simulink model "RCAM_SIMULATION"  (R2024b)
settings: Solver=VariableStepAuto  StartTime=0.0  StopTime=1000  RelTol=1e-3
undefined symbols (not defined in the file or in its folder): RCAM_model
libraries: aerolibfltsims x2, aerolibatmos2 x1, aerolibanimutils x1, aerolibanim x1
Description:
  | RCAM [Research Civil Transport Aircraft Model]
  | 
  | To study the dynamic behaviour of the aircarft with te given control inputs.
  | , through the plots ang the animation plots using the real time simualtion.
settings Model: Creator=Rahul N  LastModifiedBy=rukky
settings DataIOCC: SaveTime=off  ReturnWorkspaceOutputs=off
settings ModelReferenceCC: EnableRefExpFcnMdlSchedulingChecks=on
settings RTWCC: GPUComputeCapability=3.5

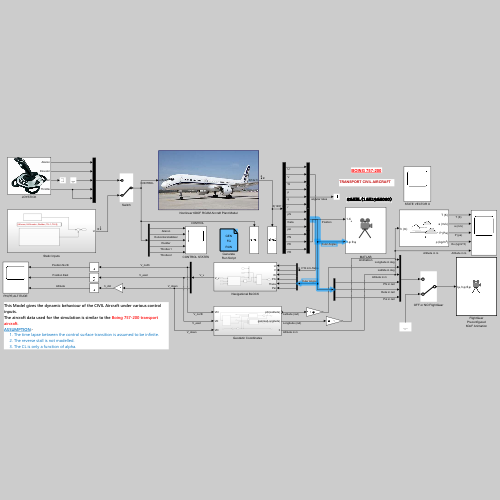
[thumbnail: Simulink's stored preview of the top-level diagram]
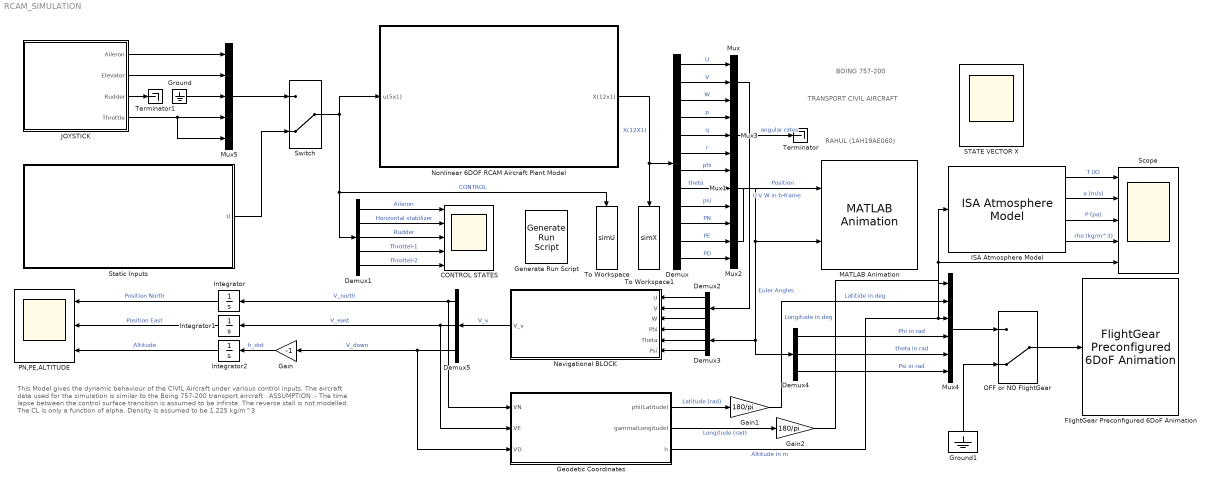
== system RCAM_SIMULATION ==
  note: RAHUL (1AH19AE060)
  note: This Model gives the dynamic behaviour of the CIVIL Aircraft under various control inputs.
      | The aircraft data used for the simulation is similar to the Boing 757-200 transport aircraft .
      | ASSUMPTION :-
      | The time lapse between the control surface transition is assumed to be infinite.
      | The reverse stall is not modelled.
      | The CL is only a function of alpha.
      | Density is assumed to be 1.225 kg/m^3
  note: TRANSPORT CIVIL AIRCRAFT
  note: BOING 757-200
  "CONTROL STATES " : Scope  NumInputPorts=5
  Demux : Demux  Outputs=12
  Demux1 : Demux  Outputs=5
  Demux{2..5} (4 alike) : Demux  Outputs=3
  FlightGear Preconfigured 6DoF Animation : aerolibfltsims/FlightGear Preconfigured 6DoF Animation  xFlightGearVersion=v2019.1  DestinationIpAddress=127.0.0.1  DestinationPort=5502  SampleTime=1/30  packetVersion=24
  Gain : Gain  Gain=-1
  Gain1 : Gain  Gain=180/pi
  Gain2 : Gain  Gain=180/pi
  Generate Run Script : aerolibfltsims/Generate Run Script  Architecture=Win64  dataFlow=Send  GeometryModelName=c172p  AirportId=KSFO  RunwayId=10L  InitialAltitude=7224  InitialHeading=113  OffsetDistance=4.72  OffsetAzimuth=0  InstallScenery=off  DisableShaders=on  OriginAddress=127.0.0.1  DestinationPort=5502  OriginPort=5505  LocalAddress=127.0.0.1  OutputFileName=runfg.bat  FlightGearBaseDirectory=C:\Program Files\FlightGear 2020.3
  Geodetic Coordinates : Subsystem
  Ground : Ground
  Ground1 : Ground
  ISA Atmosphere Model : aerolibatmos2/ISA Atmosphere Model  useExtended=off  action=Warning  custom=off  viscosityOut=off  g=9.80665  gamma=1.4  R=287.0531  L=0.0065  h_trop=11000  h_strat=20000  rho0=1.225  P0=101325  T0=288.15  h0=0  S=110.4  Tref=273.15  muref=1.716e-5
  Integrator : Integrator
  Integrator1 : Integrator
  Integrator2 : Integrator  InitialCondition=150
  JOYSTICK : Subsystem
      mask Display: image('$imagefile'); % Use "Edit Image" on toolstrip to change.
  MATLAB Animation : aerolibanim/MATLAB Animation  Tag=Matlab Animation 6 DOF  Vehicles=1  Geometries='pa24-250_orange.ac'  BoundingBoxCoordinates=[-50,50,-50,50,-50,50]  CameraOffset=[-150,-50,0]  CameraViewAngle=3  SampleTime=0.2  FigurePosition=[1,49,1280,7.033333e+02]
  Mux{,1..3} (4 alike) : Mux  Inputs=3
  Mux4 : Mux  Inputs=6
  Mux5 : Mux  Inputs=5
  Navigational BLOCK : Subsystem
  Nonlinear 6DOF RCAM Aircraft Plant Model : Subsystem
      mask Display: image('$imagefile'); % Use "Edit Image" on toolstrip to change.
  OFF or NO FlightGear : ManualSwitch  CurrentSetting=0
  PN,PE,ALTITUDE : Scope  NumInputPorts=3
  STATE VECTOR X : Scope
      settings: Floating=on
  Scope : Scope  NumInputPorts=5
  Static Inputs : Subsystem
  Switch : ManualSwitch  CurrentSetting=0
  Terminator : Terminator
  Terminator1 : Terminator
  To Workspace : ToWorkspace  VariableName=simU  SaveFormat=Timeseries  SampleTime=-1
  To Workspace1 : ToWorkspace  VariableName=simX  SaveFormat=Timeseries  SampleTime=-1
  wires:
  Demux1/1 -> "CONTROL STATES "/1  "Aileron"
  Demux1/2 -> "CONTROL STATES "/2  "Horizontal stabilizer"
  Demux1/3 -> "CONTROL STATES "/3  "Rudder"
  Demux1/4 -> "CONTROL STATES "/4  "Throttel-1"
  Demux1/5 -> "CONTROL STATES "/5  "Throttel-2"
  Switch/1 -> Nonlinear 6DOF RCAM Aircraft Plant Model/1(u(5x1)), To Workspace/1, Demux1/1  "CONTROL"
  Nonlinear 6DOF RCAM Aircraft Plant Model/1(X(12x1)) -> To Workspace1/1, Demux/1  "X(12X1)"
  Demux5/3 -> Gain/1, Geodetic Coordinates/3(VD)  "V_down"
  Gain/1 -> Integrator2/1  "h_dot"
  Integrator/1 -> PN,PE,ALTITUDE/1  "Position North"
  Demux5/1 -> Geodetic Coordinates/1(VN), Integrator/1  "V_north"
  Integrator1/1 -> PN,PE,ALTITUDE/2  "Position East"
  Integrator2/1 -> PN,PE,ALTITUDE/3  "Altitude"
  Demux5/2 -> Geodetic Coordinates/2(VE), Integrator1/1  "V_east"
  Navigational BLOCK/1(V_v) -> Demux5/1  "V_v"
  Demux/1 -> Mux/1  "U"
  Demux/2 -> Mux/2  "V"
  Demux/3 -> Mux/3  "W"
  Demux2/1 -> Navigational BLOCK/1(U)
  Demux2/2 -> Navigational BLOCK/2(V)
  Demux2/3 -> Navigational BLOCK/3(W)
  Mux/1 -> Demux2/1  "U V W in b-frame"
  Demux3/2 -> Navigational BLOCK/5(Theta)
  Demux3/3 -> Navigational BLOCK/6(Psi)
  Demux3/1 -> Navigational BLOCK/4(Phi)
  Demux/7 -> Mux1/1  "phi"
  Demux/8 -> Mux1/2  "theta"
  Demux/9 -> Mux1/3  "psi"
  Mux1/1 -> Demux4/1, Demux3/1, MATLAB Animation/2  "Euler Angles"
  Demux/10 -> Mux2/1  "PN"
  Demux/11 -> Mux2/2  "PE"
  Demux/12 -> Mux2/3  "PD"
  Demux/4 -> Mux3/1  "p"
  Demux/5 -> Mux3/2  "q"
  Demux/6 -> Mux3/3  "r"
  Mux3/1 -> Terminator/1  "angular rates"
  Geodetic Coordinates/2(gamma(Longitude)) -> Gain2/1  "Longitude (rad)"
  Gain2/1 -> Mux4/1  "Longitude in deg"
  Gain1/1 -> Mux4/2  "Latitide in deg"
  Geodetic Coordinates/3(h) -> Scope/5, ISA Atmosphere Model/1, Mux4/3  "Altitude in m"
  Demux4/1 -> Mux4/4  "Phi in rad"
  Demux4/2 -> Mux4/5  "theta in rad"
  Demux4/3 -> Mux4/6  "Psi in rad"
  Geodetic Coordinates/1(phi(Latitude)) -> Gain1/1  "Latitude (rad)"
  JOYSTICK/4(Throttle) -> Mux5/5, Mux5/4
  JOYSTICK/2(Elevator) -> Mux5/2
  JOYSTICK/1(Aileron) -> Mux5/1
  JOYSTICK/3(Rudder) -> Terminator1/1
  Ground/1 -> Mux5/3
  Mux5/1 -> Switch/1
  Static Inputs/1(U) -> Switch/2
  Mux2/1 -> MATLAB Animation/1  "Position"
  OFF or NO FlightGear/1 -> FlightGear Preconfigured 6DoF Animation/1
  Mux4/1 -> OFF or NO FlightGear/1
  Ground1/1 -> OFF or NO FlightGear/2
  ISA Atmosphere Model/1 -> Scope/1  "T (K)"
  ISA Atmosphere Model/2 -> Scope/2  "a (m/s)"
  ISA Atmosphere Model/3 -> Scope/3  "P (pa)"
  ISA Atmosphere Model/4 -> Scope/4  "rho (kg/m^3)"

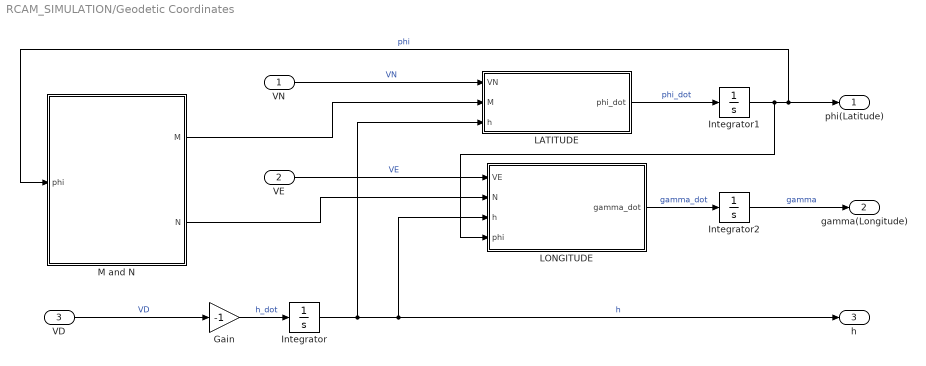
== system RCAM_SIMULATION/Geodetic Coordinates ==
  VN : Inport
  VE : Inport  Port=2
  VD : Inport  Port=3
  Gain : Gain  Gain=-1
  Integrator : Integrator  InitialCondition=150
  Integrator1 : Integrator  InitialCondition=0.22181
  Integrator2 : Integrator  InitialCondition=1.356068
  LATITUDE : MATLAB Function  TreatAsAtomicUnit=on
  LONGITUDE : MATLAB Function  TreatAsAtomicUnit=on
  M and N : Subsystem
  phi(Latitude) : Outport
  gamma(Longitude) : Outport  Port=2
  h : Outport  Port=3
  wires:
  VD/1 -> Gain/1  "VD"
  Gain/1 -> Integrator/1  "h_dot"
  Integrator/1 -> LATITUDE/3(h), LONGITUDE/3(h), h/1  "h"
  M and N/1(M) -> LATITUDE/2(M)
  M and N/2(N) -> LONGITUDE/2(N)
  LATITUDE/1(phi_dot) -> Integrator1/1  "phi_dot"
  Integrator1/1 -> LONGITUDE/4(phi), M and N/1(phi), phi(Latitude)/1  "phi"
  VE/1 -> LONGITUDE/1(VE)  "VE"
  VN/1 -> LATITUDE/1(VN)  "VN"
  LONGITUDE/1(gamma_dot) -> Integrator2/1  "gamma_dot"
  Integrator2/1 -> gamma(Longitude)/1  "gamma"

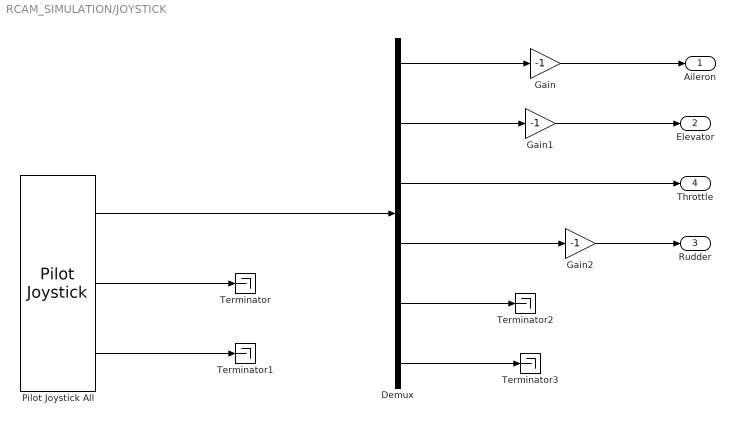
== system RCAM_SIMULATION/JOYSTICK ==
  Demux : Demux  Outputs=6
  Gain : Gain  Gain=-1
  Gain1 : Gain  Gain=-1
  Gain2 : Gain  Gain=-1
  Pilot Joystick All : aerolibanimutils/Pilot Joystick  JoystickID=None  OutputConfiguration=AllOutputs  SampleTime=1/30
  Terminator{,1..3} (4 alike) : Terminator
  Aileron : Outport
  Elevator : Outport  Port=2
  Rudder : Outport  Port=3
  Throttle : Outport  Port=4
  wires:
  Pilot Joystick All/1 -> Demux/1
  Pilot Joystick All/2 -> Terminator/1
  Pilot Joystick All/3 -> Terminator1/1
  Demux/3 -> Throttle/1
  Demux/1 -> Gain/1
  Gain/1 -> Aileron/1
  Demux/2 -> Gain1/1
  Gain1/1 -> Elevator/1
  Demux/4 -> Gain2/1
  Gain2/1 -> Rudder/1
  Demux/5 -> Terminator2/1
  Demux/6 -> Terminator3/1

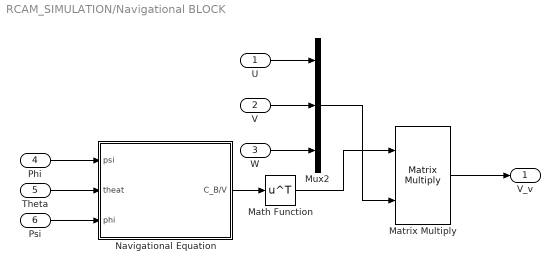
== system RCAM_SIMULATION/Navigational BLOCK ==
  U : Inport
  V : Inport  Port=2
  W : Inport  Port=3
  Phi : Inport  Port=4
  Theta : Inport  Port=5
  Psi : Inport  Port=6
  Math Function : Math  Operator=transpose
  Matrix Multiply : Product  Multiplication=Matrix(*)
  Mux2 : Mux  Inputs=3
  Navigational Equation : Subsystem
  V_v : Outport
  wires:
  V/1 -> Mux2/2
  Psi/1 -> Navigational Equation/3(phi)
  W/1 -> Mux2/3
  Navigational Equation/1(C_B/V) -> Math Function/1
  Matrix Multiply/1 -> V_v/1
  Theta/1 -> Navigational Equation/2(theat)
  U/1 -> Mux2/1
  Phi/1 -> Navigational Equation/1(psi)
  Math Function/1 -> Matrix Multiply/1
  Mux2/1 -> Matrix Multiply/2

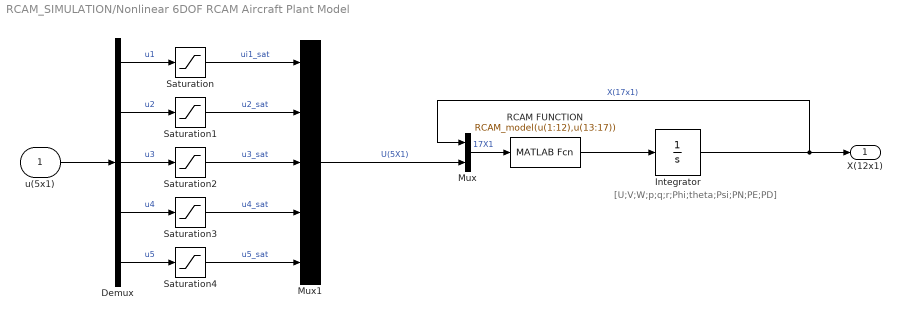
== system RCAM_SIMULATION/Nonlinear 6DOF RCAM Aircraft Plant Model ==
  note: [U;V;W;p;q;r;Phi;theta;Psi;PN;PE;PD]
  u(5x1) : Inport
  Demux : Demux  Outputs=5
  Integrator : Integrator  InitialCondition=|
      | [84.9905; 0;
      |  1.2713;
      | 0; 0; 0; 0; 0.1; 0; 0; 0.0149; 0]
  Mux : Mux  Inputs=2
  Mux1 : Mux  Inputs=5
  RCAM FUNCTION : MATLABFcn  MATLABFcn=RCAM_model(u(1:12),u(13:17))
  Saturation : Saturate  UpperLimit=25*(pi/180)  LowerLimit=-15*(pi/180)
  Saturation1 : Saturate  UpperLimit=10*(pi/180)  LowerLimit=-25*(pi/180)
  Saturation2 : Saturate  UpperLimit=30*(pi/180)  LowerLimit=-30*(pi/180)
  Saturation3 : Saturate  UpperLimit=10*(pi/180)  LowerLimit=0.5*(pi/180)
  Saturation4 : Saturate  UpperLimit=10*(pi/180)  LowerLimit=0.5*(pi/180)
  X(12x1) : Outport
  wires:
  Integrator/1 -> Mux/1, X(12x1)/1  "X(17x1)"
  u(5x1)/1 -> Demux/1
  Demux/1 -> Saturation/1  "u1"
  Saturation/1 -> Mux1/1  "ui1_sat"
  Demux/2 -> Saturation1/1  "u2"
  Demux/3 -> Saturation2/1  "u3"
  Demux/4 -> Saturation3/1  "u4"
  Demux/5 -> Saturation4/1  "u5"
  Saturation1/1 -> Mux1/2  "u2_sat"
  Saturation2/1 -> Mux1/3  "u3_sat"
  Saturation3/1 -> Mux1/4  "u4_sat"
  Saturation4/1 -> Mux1/5  "u5_sat"
  RCAM FUNCTION/1 -> Integrator/1
  Mux/1 -> RCAM FUNCTION/1  "17X1"
  Mux1/1 -> Mux/2  "U(5X1)"

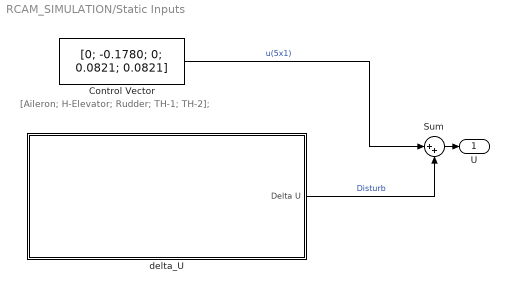
== system RCAM_SIMULATION/Static Inputs ==
  note: [Aileron; H-Elevator; Rudder; TH-1; TH-2];
  Control Vector : Constant  Value=[0; -0.1780; 0; 0.0821; 0.0821]
  Sum : Sum  Inputs=|++
  delta_U : Subsystem
  U : Outport
  wires:
  Control Vector/1 -> Sum/1  "u(5x1)"
  delta_U/1(Delta U) -> Sum/2  "Disturb"
  Sum/1 -> U/1

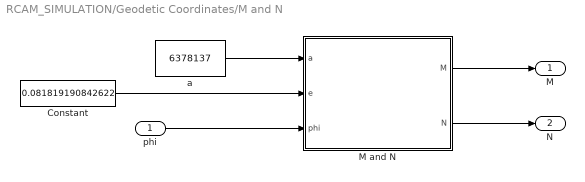
== system RCAM_SIMULATION/Geodetic Coordinates/M and N ==
  phi : Inport
  Constant : Constant  Value=0.081819190842622
  M and N : MATLAB Function  TreatAsAtomicUnit=on
  a : Constant  Value=6378137
  M : Outport
  N : Outport  Port=2
  wires:
  Constant/1 -> M and N/2(e)
  phi/1 -> M and N/3(phi)
  M and N/1(M) -> M/1
  a/1 -> M and N/1(a)
  M and N/2(N) -> N/1

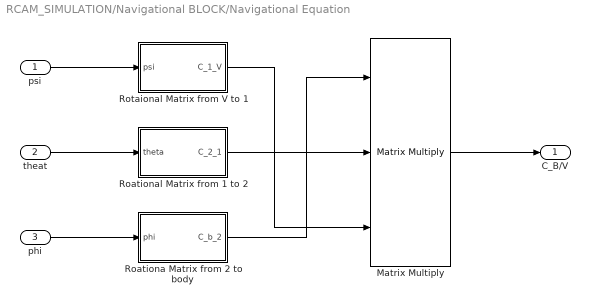
== system RCAM_SIMULATION/Navigational BLOCK/Navigational Equation ==
  psi : Inport
  theat : Inport  Port=2
  phi : Inport  Port=3
  Matrix Multiply : Product  Inputs=3  Multiplication=Matrix(*)
  Roationa Matrix from 2 to body : MATLAB Function  TreatAsAtomicUnit=on
  Roational Matrix from 1 to 2 : MATLAB Function  TreatAsAtomicUnit=on
  Rotaional Matrix from V to 1 : MATLAB Function  TreatAsAtomicUnit=on
  C_B/V : Outport
  wires:
  psi/1 -> Rotaional Matrix from V to 1/1(psi)
  theat/1 -> Roational Matrix from 1 to 2/1(theta)
  phi/1 -> Roationa Matrix from 2 to body/1(phi)
  Roationa Matrix from 2 to body/1(C_b_2) -> Matrix Multiply/1
  Roational Matrix from 1 to 2/1(C_2_1) -> Matrix Multiply/2
  Rotaional Matrix from V to 1/1(C_1_V) -> Matrix Multiply/3
  Matrix Multiply/1 -> C_B/V/1

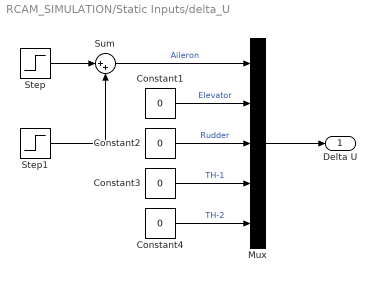
== system RCAM_SIMULATION/Static Inputs/delta_U ==
  Constant{1..4} (4 alike) : Constant  Value=0
  Mux : Mux  Inputs=5
  Step : Step  Time=15  After=10*(pi/180)  SampleTime=0
  Step1 : Step  Time=15+5  After=-10*(pi/180)  SampleTime=0
  Sum : Sum  Inputs=|++
  Delta U : Outport
  wires:
  Mux/1 -> Delta U/1
  Constant4/1 -> Mux/5  "TH-2"
  Constant2/1 -> Mux/3  "Rudder"
  Constant3/1 -> Mux/4  "TH-1"
  Constant1/1 -> Mux/2  "Elevator"
  Sum/1 -> Mux/1  "Aileron"
  Step/1 -> Sum/1
  Step1/1 -> Sum/2

== matlab function RCAM_SIMULATION/Navigational BLOCK/Navigational Equation/Roational Matrix from 1 to 2 ==
  data: theta input; C_2_1 output
function C_2_1 = fcn(theta)

% Roational Matrix From the 1 frame to 2 frame

C_2_1=[cos(theta) 0 -sin(theta); 0 1 0; sin(theta) 0 cos(theta)];

end

== matlab function RCAM_SIMULATION/Navigational BLOCK/Navigational Equation/Rotaional Matrix from V to 1 ==
  data: psi input; C_1_V output
function C_1_V = fcn(psi)

% Calculating the Rotaional Matrix  from the NED to 1 frame

C_1_V=[cos(psi) sin(psi) 0; -sin(psi) cos(psi) 0; 0 0 1];

end

== matlab function RCAM_SIMULATION/Navigational BLOCK/Navigational Equation/Roationa Matrix from 2 to body ==
  data: phi input; C_b_2 output
function C_b_2 = fcn(phi)

% Roational Matrix from the 2 frame to body frame
C_b_2=[1 0 0; 0 cos(phi) sin(phi); 0 -sin(phi) cos(phi)];
end

== matlab function RCAM_SIMULATION/Geodetic Coordinates/M and N/M and N ==
  data: a input; M output; e input; phi input; N output
function[M,N]=M_N(a,e,phi)

M=(a*(1-e*2)/(1-(e^2)*sin(phi))^3/2);  % Meridian Radius of Curvature

N=a/(1-(e^2)*(sin(phi)^2))^3/2;        % Prime verical radius of curvature

end

== matlab function RCAM_SIMULATION/Geodetic Coordinates/LATITUDE ==
  data: VN input; phi_dot output; M input; h input
function phi_dot =Latitude_Rate(VN,M,h)
% Calculating the Rate of change of Latitude

phi_dot=VN/(M+h);
end

== matlab function RCAM_SIMULATION/Geodetic Coordinates/LONGITUDE ==
  data: VE input; gamma_dot output; N input; h input; phi input
function gamma_dot =Longitude_Rate(VE,N,h,phi)

% Calculating the Rate of change of the Longitude

gamma_dot=VE/((N+h)*cos(phi));
end
